simulink model "lab6_task3"  (R2024b)
settings: Solver=ode45  StartTime=0.0  StopTime=5.0  MaxStep=0.01  RelTol=1e-3
settings Model: Creator=Beanie  LastModifiedBy=Beanie

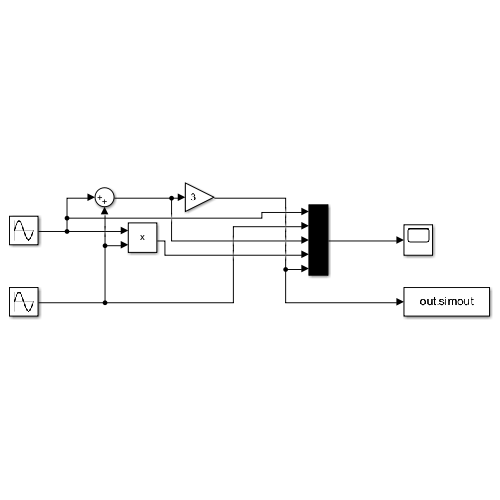
[thumbnail: Simulink's stored preview of the top-level diagram]
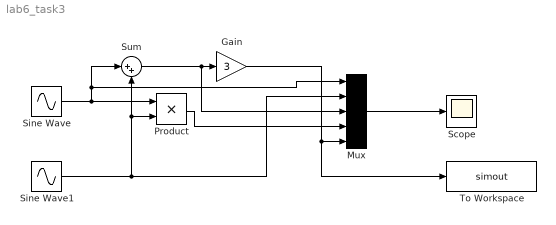
== system lab6_task3 ==
  Gain : Gain  Gain=3
  Mux : Mux  Inputs=5
  Product : Product
  Scope : Scope
  Sine Wave : Sin  Amplitude=2  Frequency=2*pi  SampleTime=0
  Sine Wave1 : Sin  Frequency=8*pi  SampleTime=0
  Sum : Sum  Inputs=|++
  To Workspace : ToWorkspace  VariableName=simout  SaveFormat=Structure With Time  SampleTime=-1
  wires:
  Sine Wave/1 -> Product/1, Sum/1, Mux/1
  Sine Wave1/1 -> Mux/2, Product/2, Sum/2
  Sum/1 -> Mux/3, Gain/1
  Mux/1 -> Scope/1
  Product/1 -> Mux/4
  Gain/1 -> To Workspace/1, Mux/5
